simulink library "xps_library"  (Simulink 8.0)
settings: Solver=ode45  SolverMode=SingleTasking  StartTime=0.0  StopTime=10.0  RelTol=1e-3
undefined symbols (not defined in the file): sys_clk, xps_library_software_register_user_data_in
libraries: xbsIndex_r4 x867, simulink x109, dspsigops x81, casper_library_flow_control x68, xps_library x18, casper_library_misc x11
(part 7 of 10)

== system xps_library/Shared BRAM/mem ==
  note: Undo address
      | manipulation for
      | simulated data
  note: Undo data manipulation on way in and redo on way out for simulated data
  In1 : Inport
  In2 : Inport  Port=2
  In3 : Inport  Port=3
  Disregard Subsystem : xbsIndex_r4/Disregard Subsystem  Tag=discardX  block_type=disregard
  calc_add : Subsystem  mask{data_width=32, addr_width=10, sample_rate=sample_rate}
      mask prompts: data_width "data width"; addr_width "address width"; sample_rate "sample rate"
  ram : xbsIndex_r4/Single Port RAM  depth=2^addr_width  initVector=init_vals  distributed_mem=Block RAM  write_mode=Read After Write  rst=off  init_reg=0  en=off  latency=1  dbl_ovrd=off  optimize=Area  block_type=spram
  sim_addr : xbsIndex_r4/Gateway In  gui_display_data_type=Fixed-point  arith_type=Unsigned  n_bits=addr_width  bin_pt=0  preci_type=Single  exp_width=8  frac_width=24  quantization=Truncate  overflow=Wrap  period=sample_rate  dbl_ovrd=off  timing_constraint=None  locs_specified=off  LOCs={}  hdl_port=on  block_type=gatewayin
      settings: infoedit="Gateway in block.  Converts inputs of type Simulink integer, double and fixed point to  Xilinx fixed point type.<br><br>Hardware notes:  In hardware these blocks become top level input ports."  xl_area=[0, 0, 0, 0, 0, 0, 0]  sginterface={'Nallatech'=>{'xdspkit'=>{'non_memory_mapped_port'=>'sim_addr'}},'Xilinx'=>{'jtaghwcosim'=>{'non_memory_mapped_port'=>'sim_addr'},'xdspkit'=>{'non_memory_mapped_port'=>'sim_addr'}}}
  sim_data_in : xbsIndex_r4/Gateway In  gui_display_data_type=Fixed-point  arith_type=Unsigned  n_bits=32  bin_pt=0  preci_type=Single  exp_width=8  frac_width=24  quantization=Truncate  overflow=Wrap  period=sample_rate  dbl_ovrd=off  timing_constraint=None  locs_specified=off  LOCs={}  hdl_port=on  block_type=gatewayin
      settings: xl_area=[0, 0, 0, 0, 0, 0, 0]  sginterface={'Nallatech'=>{'xdspkit'=>{'non_memory_mapped_port'=>'sim_data_in'}},'Xilinx'=>{'jtaghwcosim'=>{'non_memory_mapped_port'=>'sim_data_in'},'xdspkit'=>{'non_memory_mapped_port'=>'sim_data_in'}}}
  sim_data_out : xbsIndex_r4/Gateway Out  hdl_port=on  timing_constraint=None  locs_specified=off  LOCs={'B21','B22','A22','B23','B19','C19','A20','A21','A23','B24','A24','A25','E18','D18','C18','B18'}  block_type=gatewayout
      settings: infoedit="Gateway out block.  Converts Xilinx fixed point inputs into ouputs of type Simulink integer, double, or fixed point.<P><P>Hardware notes:  In hardware these blocks become top level output ports or are discarded, depending on how they are configured."  xl_area=[0, 0, 0, 0, 0, 0, 0]  sginterface={'Nallatech'=>{'xdspkit'=>{'non_memory_mapped_port'=>'sim_data_out'}},'Xilinx'=>{'jtaghwcosim'=>{'non_memory_mapped_port'=>'sim_data_out'},'xdspkit'=>{'non_memory_mapped_port'=>'sim_data_out'}}}
  sim_munge_in : Subsystem  AncestorBlock=casper_library_flow_control/munge  mask(munge){divisions=1, div_size=32, order=[0], arith_type_out=Unsigned, bin_pt_out=0}
      mask prompts: divisions "Number of divisions"; div_size "Division size (bits)"; order "Division packing order"; arith_type_out "Output arithmetic type"; bin_pt_out "Output binary point"
      mask help: Splits an input bus into the specified number of divisions and then recombines them in the order specified (most significant division = 0,least = number divisions-1)
      mask init:
      | munge_init(gcb, ...
      |     'divisions', divisions, ...
      |     'div_size', div_size, ...
      |     'order', order, ...
      |     'arith_type_out', arith_type_out, ...
      |     'bin_pt_out', bin_pt_out);
      settings: AttributesFormatString=|
      | split:32
      | join:0
      | Unsigned [32,0]
      mask TypeOptions arith_type_out: Unsigned | Signed  (2's comp) | Floating-point
  sim_munge_out : Subsystem  AncestorBlock=casper_library_flow_control/munge  mask(munge){divisions=1, div_size=32, order=[0], arith_type_out=Unsigned, bin_pt_out=0}
      mask prompts: divisions "Number of divisions"; div_size "Division size (bits)"; order "Division packing order"; arith_type_out "Output arithmetic type"; bin_pt_out "Output binary point"
      mask help: Splits an input bus into the specified number of divisions and then recombines them in the order specified (most significant division = 0,least = number divisions-1)
      mask init:
      | munge_init(gcb, ...
      |     'divisions', divisions, ...
      |     'div_size', div_size, ...
      |     'order', order, ...
      |     'arith_type_out', arith_type_out, ...
      |     'bin_pt_out', bin_pt_out);
      settings: AttributesFormatString=|
      | split:32
      | join:0
      | Unsigned [32,0]
      mask TypeOptions arith_type_out: Unsigned | Signed  (2's comp) | Floating-point
  sim_we : xbsIndex_r4/Gateway In  gui_display_data_type=Fixed-point  arith_type=Boolean  n_bits=1  bin_pt=0  preci_type=Single  exp_width=8  frac_width=24  quantization=Truncate  overflow=Wrap  period=sample_rate  dbl_ovrd=off  timing_constraint=None  locs_specified=off  LOCs={}  hdl_port=on  block_type=gatewayin
      settings: infoedit="Gateway in block.  Converts inputs of type Simulink integer, double and fixed point to  Xilinx fixed point type.<br><br>Hardware notes:  In hardware these blocks become top level input ports."  xl_area=[0, 0, 0, 0, 0, 0, 0]  sginterface={'Nallatech'=>{'xdspkit'=>{'non_memory_mapped_port'=>'sim_we'}},'Xilinx'=>{'jtaghwcosim'=>{'non_memory_mapped_port'=>'sim_we'},'xdspkit'=>{'non_memory_mapped_port'=>'sim_we'}}}
  Out1 : Outport
  wires:
  sim_munge_in/1(dout) -> ram/2
  ram/1 -> sim_munge_out/1(din)
  sim_we/1 -> ram/3
  sim_data_in/1 -> sim_munge_in/1(din)
  sim_addr/1 -> calc_add/1(in)
  In3/1 -> sim_we/1
  sim_data_out/1 -> Out1/1
  In2/1 -> sim_data_in/1
  In1/1 -> sim_addr/1
  sim_munge_out/1(dout) -> sim_data_out/1
  calc_add/1(out) -> ram/1

== system xps_library/Shared BRAM/munge_in ==
  din : Inport
  reinterpret_out : xbsIndex_r4/Reinterpret  force_arith_type=on  arith_type=Unsigned  force_bin_pt=on  bin_pt=0  block_type=reinterpret
  dout : Outport
  wires:
  reinterpret_out/1 -> dout/1
  din/1 -> reinterpret_out/1

== system xps_library/Shared BRAM/munge_out ==
  din : Inport
  reinterpret_out : xbsIndex_r4/Reinterpret  force_arith_type=on  arith_type=Unsigned  force_bin_pt=on  bin_pt=0  block_type=reinterpret
  dout : Outport
  wires:
  reinterpret_out/1 -> dout/1
  din/1 -> reinterpret_out/1

== system xps_library/adc/conv ==
  In1 : Inport
  Concat : xbsIndex_r4/Concat  num_inputs=2  dbl_ovrd=off  block_type=concat
      settings: block_version=8.2.02
  Inverter : xbsIndex_r4/Inverter  en=off  latency=0  dbl_ovrd=off  block_type=inv
      settings: xl_area=[0, 0, 0, 0, 0, 0, 0]  block_version=8.2.02
  Reinterpret : xbsIndex_r4/Reinterpret  force_arith_type=on  arith_type="Signed  (2's comp)"  force_bin_pt=on  bin_pt=7  block_type=reinterpret
      settings: infoedit="Changes signal type without altering the binary representation.   You can changed the signal between signed and unsigned, and relocate the binary point.<P><P>Hardware notes: In hardware this block costs nothing.<P><P>Example:  Suppose the input is 6 bits wide, signed, with 2 fractional bits, and the output is forced to unsigned with 0 fractional bits.  Then an input of -2.0 (1110.00 in binary 2's complement) becomes an output of 56 (111000 in binary)."  block_version=8.2.02
  Slice : xbsIndex_r4/Slice  nbits=1  boolean_output=off  mode=Upper Bit Location + Width  bit1=0  base1=MSB of Input  bit0=0  base0=LSB of Input  dbl_ovrd=off  block_type=slice
      settings: infoedit="Extracts a given range of bits from each input sample and presents it at the output.  The output type is ordinarily unsigned with binary point at zero, but can be Boolean when the slice is one bit wide.<P><P>Hardware notes: In hardware this block costs nothing."  block_version=8.2.02
  Slice1 : xbsIndex_r4/Slice  nbits=7  boolean_output=off  mode=Lower Bit Location + Width  bit1=0  base1=MSB of Input  bit0=0  base0=LSB of Input  dbl_ovrd=off  block_type=slice
      settings: infoedit="Extracts a given range of bits from each input sample and presents it at the output.  The output type is ordinarily unsigned with binary point at zero, but can be Boolean when the slice is one bit wide.<P><P>Hardware notes: In hardware this block costs nothing."  block_version=8.2.02
  Out1 : Outport
  wires:
  Reinterpret/1 -> Out1/1
  Concat/1 -> Reinterpret/1
  Slice1/1 -> Concat/2
  Inverter/1 -> Concat/1
  Slice/1 -> Inverter/1
  In1/1 -> Slice/1, Slice1/1

== system xps_library/adc/conv1 ==
  In1 : Inport
  Concat : xbsIndex_r4/Concat  num_inputs=2  dbl_ovrd=off  block_type=concat
      settings: block_version=8.2.02
  Inverter : xbsIndex_r4/Inverter  en=off  latency=0  dbl_ovrd=off  block_type=inv
      settings: xl_area=[0, 0, 0, 0, 0, 0, 0]  block_version=8.2.02
  Reinterpret : xbsIndex_r4/Reinterpret  force_arith_type=on  arith_type="Signed  (2's comp)"  force_bin_pt=on  bin_pt=7  block_type=reinterpret
      settings: infoedit="Changes signal type without altering the binary representation.   You can changed the signal between signed and unsigned, and relocate the binary point.<P><P>Hardware notes: In hardware this block costs nothing.<P><P>Example:  Suppose the input is 6 bits wide, signed, with 2 fractional bits, and the output is forced to unsigned with 0 fractional bits.  Then an input of -2.0 (1110.00 in binary 2's complement) becomes an output of 56 (111000 in binary)."  block_version=8.2.02
  Slice : xbsIndex_r4/Slice  nbits=1  boolean_output=off  mode=Upper Bit Location + Width  bit1=0  base1=MSB of Input  bit0=0  base0=LSB of Input  dbl_ovrd=off  block_type=slice
      settings: infoedit="Extracts a given range of bits from each input sample and presents it at the output.  The output type is ordinarily unsigned with binary point at zero, but can be Boolean when the slice is one bit wide.<P><P>Hardware notes: In hardware this block costs nothing."  block_version=8.2.02
  Slice1 : xbsIndex_r4/Slice  nbits=7  boolean_output=off  mode=Lower Bit Location + Width  bit1=0  base1=MSB of Input  bit0=0  base0=LSB of Input  dbl_ovrd=off  block_type=slice
      settings: infoedit="Extracts a given range of bits from each input sample and presents it at the output.  The output type is ordinarily unsigned with binary point at zero, but can be Boolean when the slice is one bit wide.<P><P>Hardware notes: In hardware this block costs nothing."  block_version=8.2.02
  Out1 : Outport
  wires:
  Reinterpret/1 -> Out1/1
  Concat/1 -> Reinterpret/1
  Slice1/1 -> Concat/2
  Inverter/1 -> Concat/1
  Slice/1 -> Inverter/1
  In1/1 -> Slice/1, Slice1/1

== system xps_library/adc/conv2 ==
  In1 : Inport
  Concat : xbsIndex_r4/Concat  num_inputs=2  dbl_ovrd=off  block_type=concat
      settings: block_version=8.2.02
  Inverter : xbsIndex_r4/Inverter  en=off  latency=0  dbl_ovrd=off  block_type=inv
      settings: xl_area=[0, 0, 0, 0, 0, 0, 0]  block_version=8.2.02
  Reinterpret : xbsIndex_r4/Reinterpret  force_arith_type=on  arith_type="Signed  (2's comp)"  force_bin_pt=on  bin_pt=7  block_type=reinterpret
      settings: infoedit="Changes signal type without altering the binary representation.   You can changed the signal between signed and unsigned, and relocate the binary point.<P><P>Hardware notes: In hardware this block costs nothing.<P><P>Example:  Suppose the input is 6 bits wide, signed, with 2 fractional bits, and the output is forced to unsigned with 0 fractional bits.  Then an input of -2.0 (1110.00 in binary 2's complement) becomes an output of 56 (111000 in binary)."  block_version=8.2.02
  Slice : xbsIndex_r4/Slice  nbits=1  boolean_output=off  mode=Upper Bit Location + Width  bit1=0  base1=MSB of Input  bit0=0  base0=LSB of Input  dbl_ovrd=off  block_type=slice
      settings: infoedit="Extracts a given range of bits from each input sample and presents it at the output.  The output type is ordinarily unsigned with binary point at zero, but can be Boolean when the slice is one bit wide.<P><P>Hardware notes: In hardware this block costs nothing."  block_version=8.2.02
  Slice1 : xbsIndex_r4/Slice  nbits=7  boolean_output=off  mode=Lower Bit Location + Width  bit1=0  base1=MSB of Input  bit0=0  base0=LSB of Input  dbl_ovrd=off  block_type=slice
      settings: infoedit="Extracts a given range of bits from each input sample and presents it at the output.  The output type is ordinarily unsigned with binary point at zero, but can be Boolean when the slice is one bit wide.<P><P>Hardware notes: In hardware this block costs nothing."  block_version=8.2.02
  Out1 : Outport
  wires:
  Reinterpret/1 -> Out1/1
  Concat/1 -> Reinterpret/1
  Slice1/1 -> Concat/2
  Inverter/1 -> Concat/1
  Slice/1 -> Inverter/1
  In1/1 -> Slice/1, Slice1/1

== system xps_library/adc/conv3 ==
  In1 : Inport
  Concat : xbsIndex_r4/Concat  num_inputs=2  dbl_ovrd=off  block_type=concat
      settings: block_version=8.2.02
  Inverter : xbsIndex_r4/Inverter  en=off  latency=0  dbl_ovrd=off  block_type=inv
      settings: xl_area=[0, 0, 0, 0, 0, 0, 0]  block_version=8.2.02
  Reinterpret : xbsIndex_r4/Reinterpret  force_arith_type=on  arith_type="Signed  (2's comp)"  force_bin_pt=on  bin_pt=7  block_type=reinterpret
      settings: infoedit="Changes signal type without altering the binary representation.   You can changed the signal between signed and unsigned, and relocate the binary point.<P><P>Hardware notes: In hardware this block costs nothing.<P><P>Example:  Suppose the input is 6 bits wide, signed, with 2 fractional bits, and the output is forced to unsigned with 0 fractional bits.  Then an input of -2.0 (1110.00 in binary 2's complement) becomes an output of 56 (111000 in binary)."  block_version=8.2.02
  Slice : xbsIndex_r4/Slice  nbits=1  boolean_output=off  mode=Upper Bit Location + Width  bit1=0  base1=MSB of Input  bit0=0  base0=LSB of Input  dbl_ovrd=off  block_type=slice
      settings: infoedit="Extracts a given range of bits from each input sample and presents it at the output.  The output type is ordinarily unsigned with binary point at zero, but can be Boolean when the slice is one bit wide.<P><P>Hardware notes: In hardware this block costs nothing."  block_version=8.2.02
  Slice1 : xbsIndex_r4/Slice  nbits=7  boolean_output=off  mode=Lower Bit Location + Width  bit1=0  base1=MSB of Input  bit0=0  base0=LSB of Input  dbl_ovrd=off  block_type=slice
      settings: infoedit="Extracts a given range of bits from each input sample and presents it at the output.  The output type is ordinarily unsigned with binary point at zero, but can be Boolean when the slice is one bit wide.<P><P>Hardware notes: In hardware this block costs nothing."  block_version=8.2.02
  Out1 : Outport
  wires:
  Reinterpret/1 -> Out1/1
  Concat/1 -> Reinterpret/1
  Slice1/1 -> Concat/2
  Inverter/1 -> Concat/1
  Slice/1 -> Inverter/1
  In1/1 -> Slice/1, Slice1/1

== system xps_library/adc/conv4 ==
  In1 : Inport
  Concat : xbsIndex_r4/Concat  num_inputs=2  dbl_ovrd=off  block_type=concat
      settings: block_version=8.2.02
  Inverter : xbsIndex_r4/Inverter  en=off  latency=0  dbl_ovrd=off  block_type=inv
      settings: xl_area=[0, 0, 0, 0, 0, 0, 0]  block_version=8.2.02
  Reinterpret : xbsIndex_r4/Reinterpret  force_arith_type=on  arith_type="Signed  (2's comp)"  force_bin_pt=on  bin_pt=7  block_type=reinterpret
      settings: infoedit="Changes signal type without altering the binary representation.   You can changed the signal between signed and unsigned, and relocate the binary point.<P><P>Hardware notes: In hardware this block costs nothing.<P><P>Example:  Suppose the input is 6 bits wide, signed, with 2 fractional bits, and the output is forced to unsigned with 0 fractional bits.  Then an input of -2.0 (1110.00 in binary 2's complement) becomes an output of 56 (111000 in binary)."  block_version=8.2.02
  Slice : xbsIndex_r4/Slice  nbits=1  boolean_output=off  mode=Upper Bit Location + Width  bit1=0  base1=MSB of Input  bit0=0  base0=LSB of Input  dbl_ovrd=off  block_type=slice
      settings: infoedit="Extracts a given range of bits from each input sample and presents it at the output.  The output type is ordinarily unsigned with binary point at zero, but can be Boolean when the slice is one bit wide.<P><P>Hardware notes: In hardware this block costs nothing."  block_version=8.2.02
  Slice1 : xbsIndex_r4/Slice  nbits=7  boolean_output=off  mode=Lower Bit Location + Width  bit1=0  base1=MSB of Input  bit0=0  base0=LSB of Input  dbl_ovrd=off  block_type=slice
      settings: infoedit="Extracts a given range of bits from each input sample and presents it at the output.  The output type is ordinarily unsigned with binary point at zero, but can be Boolean when the slice is one bit wide.<P><P>Hardware notes: In hardware this block costs nothing."  block_version=8.2.02
  Out1 : Outport
  wires:
  Reinterpret/1 -> Out1/1
  Concat/1 -> Reinterpret/1
  Slice1/1 -> Concat/2
  Inverter/1 -> Concat/1
  Slice/1 -> Inverter/1
  In1/1 -> Slice/1, Slice1/1

== system xps_library/adc/conv5 ==
  In1 : Inport
  Concat : xbsIndex_r4/Concat  num_inputs=2  dbl_ovrd=off  block_type=concat
      settings: block_version=8.2.02
  Inverter : xbsIndex_r4/Inverter  en=off  latency=0  dbl_ovrd=off  block_type=inv
      settings: xl_area=[0, 0, 0, 0, 0, 0, 0]  block_version=8.2.02
  Reinterpret : xbsIndex_r4/Reinterpret  force_arith_type=on  arith_type="Signed  (2's comp)"  force_bin_pt=on  bin_pt=7  block_type=reinterpret
      settings: infoedit="Changes signal type without altering the binary representation.   You can changed the signal between signed and unsigned, and relocate the binary point.<P><P>Hardware notes: In hardware this block costs nothing.<P><P>Example:  Suppose the input is 6 bits wide, signed, with 2 fractional bits, and the output is forced to unsigned with 0 fractional bits.  Then an input of -2.0 (1110.00 in binary 2's complement) becomes an output of 56 (111000 in binary)."  block_version=8.2.02
  Slice : xbsIndex_r4/Slice  nbits=1  boolean_output=off  mode=Upper Bit Location + Width  bit1=0  base1=MSB of Input  bit0=0  base0=LSB of Input  dbl_ovrd=off  block_type=slice
      settings: infoedit="Extracts a given range of bits from each input sample and presents it at the output.  The output type is ordinarily unsigned with binary point at zero, but can be Boolean when the slice is one bit wide.<P><P>Hardware notes: In hardware this block costs nothing."  block_version=8.2.02
  Slice1 : xbsIndex_r4/Slice  nbits=7  boolean_output=off  mode=Lower Bit Location + Width  bit1=0  base1=MSB of Input  bit0=0  base0=LSB of Input  dbl_ovrd=off  block_type=slice
      settings: infoedit="Extracts a given range of bits from each input sample and presents it at the output.  The output type is ordinarily unsigned with binary point at zero, but can be Boolean when the slice is one bit wide.<P><P>Hardware notes: In hardware this block costs nothing."  block_version=8.2.02
  Out1 : Outport
  wires:
  Reinterpret/1 -> Out1/1
  Concat/1 -> Reinterpret/1
  Slice1/1 -> Concat/2
  Inverter/1 -> Concat/1
  Slice/1 -> Inverter/1
  In1/1 -> Slice/1, Slice1/1

== system xps_library/adc/conv6 ==
  In1 : Inport
  Concat : xbsIndex_r4/Concat  num_inputs=2  dbl_ovrd=off  block_type=concat
      settings: block_version=8.2.02
  Inverter : xbsIndex_r4/Inverter  en=off  latency=0  dbl_ovrd=off  block_type=inv
      settings: xl_area=[0, 0, 0, 0, 0, 0, 0]  block_version=8.2.02
  Reinterpret : xbsIndex_r4/Reinterpret  force_arith_type=on  arith_type="Signed  (2's comp)"  force_bin_pt=on  bin_pt=7  block_type=reinterpret
      settings: infoedit="Changes signal type without altering the binary representation.   You can changed the signal between signed and unsigned, and relocate the binary point.<P><P>Hardware notes: In hardware this block costs nothing.<P><P>Example:  Suppose the input is 6 bits wide, signed, with 2 fractional bits, and the output is forced to unsigned with 0 fractional bits.  Then an input of -2.0 (1110.00 in binary 2's complement) becomes an output of 56 (111000 in binary)."  block_version=8.2.02
  Slice : xbsIndex_r4/Slice  nbits=1  boolean_output=off  mode=Upper Bit Location + Width  bit1=0  base1=MSB of Input  bit0=0  base0=LSB of Input  dbl_ovrd=off  block_type=slice
      settings: infoedit="Extracts a given range of bits from each input sample and presents it at the output.  The output type is ordinarily unsigned with binary point at zero, but can be Boolean when the slice is one bit wide.<P><P>Hardware notes: In hardware this block costs nothing."  block_version=8.2.02
  Slice1 : xbsIndex_r4/Slice  nbits=7  boolean_output=off  mode=Lower Bit Location + Width  bit1=0  base1=MSB of Input  bit0=0  base0=LSB of Input  dbl_ovrd=off  block_type=slice
      settings: infoedit="Extracts a given range of bits from each input sample and presents it at the output.  The output type is ordinarily unsigned with binary point at zero, but can be Boolean when the slice is one bit wide.<P><P>Hardware notes: In hardware this block costs nothing."  block_version=8.2.02
  Out1 : Outport
  wires:
  Reinterpret/1 -> Out1/1
  Concat/1 -> Reinterpret/1
  Slice1/1 -> Concat/2
  Inverter/1 -> Concat/1
  Slice/1 -> Inverter/1
  In1/1 -> Slice/1, Slice1/1

== system xps_library/adc/conv7 ==
  In1 : Inport
  Concat : xbsIndex_r4/Concat  num_inputs=2  dbl_ovrd=off  block_type=concat
      settings: block_version=8.2.02
  Inverter : xbsIndex_r4/Inverter  en=off  latency=0  dbl_ovrd=off  block_type=inv
      settings: xl_area=[0, 0, 0, 0, 0, 0, 0]  block_version=8.2.02
  Reinterpret : xbsIndex_r4/Reinterpret  force_arith_type=on  arith_type="Signed  (2's comp)"  force_bin_pt=on  bin_pt=7  block_type=reinterpret
      settings: infoedit="Changes signal type without altering the binary representation.   You can changed the signal between signed and unsigned, and relocate the binary point.<P><P>Hardware notes: In hardware this block costs nothing.<P><P>Example:  Suppose the input is 6 bits wide, signed, with 2 fractional bits, and the output is forced to unsigned with 0 fractional bits.  Then an input of -2.0 (1110.00 in binary 2's complement) becomes an output of 56 (111000 in binary)."  block_version=8.2.02
  Slice : xbsIndex_r4/Slice  nbits=1  boolean_output=off  mode=Upper Bit Location + Width  bit1=0  base1=MSB of Input  bit0=0  base0=LSB of Input  dbl_ovrd=off  block_type=slice
      settings: infoedit="Extracts a given range of bits from each input sample and presents it at the output.  The output type is ordinarily unsigned with binary point at zero, but can be Boolean when the slice is one bit wide.<P><P>Hardware notes: In hardware this block costs nothing."  block_version=8.2.02
  Slice1 : xbsIndex_r4/Slice  nbits=7  boolean_output=off  mode=Lower Bit Location + Width  bit1=0  base1=MSB of Input  bit0=0  base0=LSB of Input  dbl_ovrd=off  block_type=slice
      settings: infoedit="Extracts a given range of bits from each input sample and presents it at the output.  The output type is ordinarily unsigned with binary point at zero, but can be Boolean when the slice is one bit wide.<P><P>Hardware notes: In hardware this block costs nothing."  block_version=8.2.02
  Out1 : Outport
  wires:
  Reinterpret/1 -> Out1/1
  Concat/1 -> Reinterpret/1
  Slice1/1 -> Concat/2
  Inverter/1 -> Concat/1
  Slice/1 -> Inverter/1
  In1/1 -> Slice/1, Slice1/1

== system xps_library/adc083000x2/adc_sim ==
  sim_adc_data_in : Inport
  adc_bias : Bias  Bias=128  SaturateOnIntegerOverflow=on
  adc_gain : Gain  Gain=128
  overflow_detector : Subsystem  AncestorBlock=casper_library/Misc/of_detect_bus  mask(of_detect_bus){nStreams=16, bit_width=8}
      mask prompts: nStreams "Number of Streams"; bit_width "Bit Width"
      mask init:
      | adc_overflow_detector_init(gcb, ...
      |     'nStreams', nStreams, ...
      |     'bit_width', bit_width);
  sample0_ds : dspsigops/Downsample  N=16  phase=1  smode=Force single rate  fmode=Maintain input frame rate  ic=0
  sample10_ds : dspsigops/Downsample  N=16  phase=11  smode=Force single rate  fmode=Maintain input frame rate  ic=0
  sample11_ds : dspsigops/Downsample  N=16  phase=12  smode=Force single rate  fmode=Maintain input frame rate  ic=0
  sample12_ds : dspsigops/Downsample  N=16  phase=13  smode=Force single rate  fmode=Maintain input frame rate  ic=0
  sample13_ds : dspsigops/Downsample  N=16  phase=14  smode=Force single rate  fmode=Maintain input frame rate  ic=0
  sample14_ds : dspsigops/Downsample  N=16  phase=15  smode=Force single rate  fmode=Maintain input frame rate  ic=0
  sample15_ds : dspsigops/Downsample  N=16  phase=0  smode=Force single rate  fmode=Maintain input frame rate  ic=0
  sample1_ds : dspsigops/Downsample  N=16  phase=2  smode=Force single rate  fmode=Maintain input frame rate  ic=0
  sample2_ds : dspsigops/Downsample  N=16  phase=3  smode=Force single rate  fmode=Maintain input frame rate  ic=0
  sample3_ds : dspsigops/Downsample  N=16  phase=4  smode=Force single rate  fmode=Maintain input frame rate  ic=0
  sample4_ds : dspsigops/Downsample  N=16  phase=5  smode=Force single rate  fmode=Maintain input frame rate  ic=0
  sample5_ds : dspsigops/Downsample  N=16  phase=6  smode=Force single rate  fmode=Maintain input frame rate  ic=0
  sample6_ds : dspsigops/Downsample  N=16  phase=7  smode=Force single rate  fmode=Maintain input frame rate  ic=0
  sample7_ds : dspsigops/Downsample  N=16  phase=8  smode=Force single rate  fmode=Maintain input frame rate  ic=0
  sample8_ds : dspsigops/Downsample  N=16  phase=9  smode=Force single rate  fmode=Maintain input frame rate  ic=0
  sample9_ds : dspsigops/Downsample  N=16  phase=10  smode=Force single rate  fmode=Maintain input frame rate  ic=0
  s0 : Outport
  s1 : Outport  Port=2
  s2 : Outport  Port=3
  s3 : Outport  Port=4
  s4 : Outport  Port=5
  s5 : Outport  Port=6
  s6 : Outport  Port=7
  s7 : Outport  Port=8
  s8 : Outport  Port=9
  s9 : Outport  Port=10
  s10 : Outport  Port=11
  s11 : Outport  Port=12
  s12 : Outport  Port=13
  s13 : Outport  Port=14
  s14 : Outport  Port=15
  s15 : Outport  Port=16
  of : Outport  Port=17
  wires:
  sim_adc_data_in/1 -> adc_gain/1
  adc_gain/1 -> adc_bias/1
  overflow_detector/1(overflow) -> of/1
  adc_bias/1 -> sample0_ds/1, sample1_ds/1, sample2_ds/1, sample3_ds/1, sample4_ds/1, sample5_ds/1, sample6_ds/1, sample7_ds/1, sample8_ds/1, sample9_ds/1, sample10_ds/1, sample11_ds/1, sample12_ds/1, sample13_ds/1, sample14_ds/1, sample15_ds/1
  sample0_ds/1 -> overflow_detector/1(s0), s0/1
  sample1_ds/1 -> overflow_detector/2(s1), s1/1
  sample2_ds/1 -> overflow_detector/3(s2), s2/1
  sample3_ds/1 -> overflow_detector/4(s3), s3/1
  sample4_ds/1 -> overflow_detector/5(s4), s4/1
  sample5_ds/1 -> overflow_detector/6(s5), s5/1
  sample6_ds/1 -> overflow_detector/7(s6), s6/1
  sample7_ds/1 -> overflow_detector/8(s7), s7/1
  sample8_ds/1 -> overflow_detector/9(s8), s8/1
  sample9_ds/1 -> overflow_detector/10(s9), s9/1
  sample10_ds/1 -> overflow_detector/11(s10), s10/1
  sample11_ds/1 -> overflow_detector/12(s11), s11/1
  sample12_ds/1 -> overflow_detector/13(s12), s12/1
  sample13_ds/1 -> overflow_detector/14(s13), s13/1
  sample14_ds/1 -> overflow_detector/15(s14), s14/1
  sample15_ds/1 -> overflow_detector/16(s15), s15/1

== system xps_library/adc1x1800-10/conv ==
  In1 : Inport
  Concat : xbsIndex_r4/Concat  num_inputs=2  dbl_ovrd=off  block_type=concat
      settings: block_version=8.2.02
  Inverter : xbsIndex_r4/Inverter  en=off  latency=0  dbl_ovrd=off  block_type=inv
      settings: xl_area=[0, 0, 0, 0, 0, 0, 0]  block_version=8.2.02
  Reinterpret : xbsIndex_r4/Reinterpret  force_arith_type=on  arith_type="Signed  (2's comp)"  force_bin_pt=on  bin_pt=9  block_type=reinterpret
      settings: infoedit="Changes signal type without altering the binary representation.   You can changed the signal between signed and unsigned, and relocate the binary point.<br><br>Hardware notes: In hardware this block costs nothing.<br><br>Example:  Suppose the input is 6 bits wide, signed, with 2 fractional bits, and the output is forced to unsigned with 0 fractional bits.  Then an input of -2.0 (1110.00 in binary 2's complement) becomes an output of 56 (111000 in binary)."  block_version=8.2.02
  Slice : xbsIndex_r4/Slice  nbits=1  boolean_output=off  mode=Upper Bit Location + Width  bit1=0  base1=MSB of Input  bit0=0  base0=LSB of Input  dbl_ovrd=off  block_type=slice
      settings: block_version=8.2.02
  Slice1 : xbsIndex_r4/Slice  nbits=9  boolean_output=off  mode=Lower Bit Location + Width  bit1=0  base1=MSB of Input  bit0=0  base0=LSB of Input  dbl_ovrd=off  block_type=slice
      settings: block_version=8.2.02
  Out1 : Outport
  wires:
  In1/1 -> Slice1/1, Slice/1
  Slice/1 -> Inverter/1
  Inverter/1 -> Concat/1
  Slice1/1 -> Concat/2
  Concat/1 -> Reinterpret/1
  Reinterpret/1 -> Out1/1

== system xps_library/adc1x1800-10/conv1 ==
  In1 : Inport
  Concat : xbsIndex_r4/Concat  num_inputs=2  dbl_ovrd=off  block_type=concat
      settings: block_version=8.2.02
  Inverter : xbsIndex_r4/Inverter  en=off  latency=0  dbl_ovrd=off  block_type=inv
      settings: xl_area=[0, 0, 0, 0, 0, 0, 0]  block_version=8.2.02
  Reinterpret : xbsIndex_r4/Reinterpret  force_arith_type=on  arith_type="Signed  (2's comp)"  force_bin_pt=on  bin_pt=9  block_type=reinterpret
      settings: infoedit="Changes signal type without altering the binary representation.   You can changed the signal between signed and unsigned, and relocate the binary point.<br><br>Hardware notes: In hardware this block costs nothing.<br><br>Example:  Suppose the input is 6 bits wide, signed, with 2 fractional bits, and the output is forced to unsigned with 0 fractional bits.  Then an input of -2.0 (1110.00 in binary 2's complement) becomes an output of 56 (111000 in binary)."  block_version=8.2.02
  Slice : xbsIndex_r4/Slice  nbits=1  boolean_output=off  mode=Upper Bit Location + Width  bit1=0  base1=MSB of Input  bit0=0  base0=LSB of Input  dbl_ovrd=off  block_type=slice
      settings: block_version=8.2.02
  Slice1 : xbsIndex_r4/Slice  nbits=9  boolean_output=off  mode=Lower Bit Location + Width  bit1=0  base1=MSB of Input  bit0=0  base0=LSB of Input  dbl_ovrd=off  block_type=slice
      settings: block_version=8.2.02
  Out1 : Outport
  wires:
  In1/1 -> Slice1/1, Slice/1
  Slice/1 -> Inverter/1
  Inverter/1 -> Concat/1
  Slice1/1 -> Concat/2
  Concat/1 -> Reinterpret/1
  Reinterpret/1 -> Out1/1

== system xps_library/adc1x1800-10/conv2 ==
  In1 : Inport
  Concat : xbsIndex_r4/Concat  num_inputs=2  dbl_ovrd=off  block_type=concat
      settings: block_version=8.2.02
  Inverter : xbsIndex_r4/Inverter  en=off  latency=0  dbl_ovrd=off  block_type=inv
      settings: xl_area=[0, 0, 0, 0, 0, 0, 0]  block_version=8.2.02
  Reinterpret : xbsIndex_r4/Reinterpret  force_arith_type=on  arith_type="Signed  (2's comp)"  force_bin_pt=on  bin_pt=9  block_type=reinterpret
      settings: infoedit="Changes signal type without altering the binary representation.   You can changed the signal between signed and unsigned, and relocate the binary point.<br><br>Hardware notes: In hardware this block costs nothing.<br><br>Example:  Suppose the input is 6 bits wide, signed, with 2 fractional bits, and the output is forced to unsigned with 0 fractional bits.  Then an input of -2.0 (1110.00 in binary 2's complement) becomes an output of 56 (111000 in binary)."  block_version=8.2.02
  Slice : xbsIndex_r4/Slice  nbits=1  boolean_output=off  mode=Upper Bit Location + Width  bit1=0  base1=MSB of Input  bit0=0  base0=LSB of Input  dbl_ovrd=off  block_type=slice
      settings: block_version=8.2.02
  Slice1 : xbsIndex_r4/Slice  nbits=9  boolean_output=off  mode=Lower Bit Location + Width  bit1=0  base1=MSB of Input  bit0=0  base0=LSB of Input  dbl_ovrd=off  block_type=slice
      settings: block_version=8.2.02
  Out1 : Outport
  wires:
  In1/1 -> Slice1/1, Slice/1
  Slice/1 -> Inverter/1
  Inverter/1 -> Concat/1
  Slice1/1 -> Concat/2
  Concat/1 -> Reinterpret/1
  Reinterpret/1 -> Out1/1

== system xps_library/adc1x1800-10/conv3 ==
  In1 : Inport
  Concat : xbsIndex_r4/Concat  num_inputs=2  dbl_ovrd=off  block_type=concat
      settings: block_version=8.2.02
  Inverter : xbsIndex_r4/Inverter  en=off  latency=0  dbl_ovrd=off  block_type=inv
      settings: xl_area=[0, 0, 0, 0, 0, 0, 0]  block_version=8.2.02
  Reinterpret : xbsIndex_r4/Reinterpret  force_arith_type=on  arith_type="Signed  (2's comp)"  force_bin_pt=on  bin_pt=9  block_type=reinterpret
      settings: infoedit="Changes signal type without altering the binary representation.   You can changed the signal between signed and unsigned, and relocate the binary point.<br><br>Hardware notes: In hardware this block costs nothing.<br><br>Example:  Suppose the input is 6 bits wide, signed, with 2 fractional bits, and the output is forced to unsigned with 0 fractional bits.  Then an input of -2.0 (1110.00 in binary 2's complement) becomes an output of 56 (111000 in binary)."  block_version=8.2.02
  Slice : xbsIndex_r4/Slice  nbits=1  boolean_output=off  mode=Upper Bit Location + Width  bit1=0  base1=MSB of Input  bit0=0  base0=LSB of Input  dbl_ovrd=off  block_type=slice
      settings: block_version=8.2.02
  Slice1 : xbsIndex_r4/Slice  nbits=9  boolean_output=off  mode=Lower Bit Location + Width  bit1=0  base1=MSB of Input  bit0=0  base0=LSB of Input  dbl_ovrd=off  block_type=slice
      settings: block_version=8.2.02
  Out1 : Outport
  wires:
  In1/1 -> Slice1/1, Slice/1
  Slice/1 -> Inverter/1
  Inverter/1 -> Concat/1
  Slice1/1 -> Concat/2
  Concat/1 -> Reinterpret/1
  Reinterpret/1 -> Out1/1

== system xps_library/adc1x1800-10/conv4 ==
  In1 : Inport
  Concat : xbsIndex_r4/Concat  num_inputs=2  dbl_ovrd=off  block_type=concat
      settings: block_version=8.2.02
  Inverter : xbsIndex_r4/Inverter  en=off  latency=0  dbl_ovrd=off  block_type=inv
      settings: xl_area=[0, 0, 0, 0, 0, 0, 0]  block_version=8.2.02
  Reinterpret : xbsIndex_r4/Reinterpret  force_arith_type=on  arith_type="Signed  (2's comp)"  force_bin_pt=on  bin_pt=9  block_type=reinterpret
      settings: infoedit="Changes signal type without altering the binary representation.   You can changed the signal between signed and unsigned, and relocate the binary point.<br><br>Hardware notes: In hardware this block costs nothing.<br><br>Example:  Suppose the input is 6 bits wide, signed, with 2 fractional bits, and the output is forced to unsigned with 0 fractional bits.  Then an input of -2.0 (1110.00 in binary 2's complement) becomes an output of 56 (111000 in binary)."  block_version=8.2.02
  Slice : xbsIndex_r4/Slice  nbits=1  boolean_output=off  mode=Upper Bit Location + Width  bit1=0  base1=MSB of Input  bit0=0  base0=LSB of Input  dbl_ovrd=off  block_type=slice
      settings: block_version=8.2.02
  Slice1 : xbsIndex_r4/Slice  nbits=9  boolean_output=off  mode=Lower Bit Location + Width  bit1=0  base1=MSB of Input  bit0=0  base0=LSB of Input  dbl_ovrd=off  block_type=slice
      settings: block_version=8.2.02
  Out1 : Outport
  wires:
  In1/1 -> Slice1/1, Slice/1
  Slice/1 -> Inverter/1
  Inverter/1 -> Concat/1
  Slice1/1 -> Concat/2
  Concat/1 -> Reinterpret/1
  Reinterpret/1 -> Out1/1

== system xps_library/adc1x1800-10/conv5 ==
  In1 : Inport
  Concat : xbsIndex_r4/Concat  num_inputs=2  dbl_ovrd=off  block_type=concat
      settings: block_version=8.2.02
  Inverter : xbsIndex_r4/Inverter  en=off  latency=0  dbl_ovrd=off  block_type=inv
      settings: xl_area=[0, 0, 0, 0, 0, 0, 0]  block_version=8.2.02
  Reinterpret : xbsIndex_r4/Reinterpret  force_arith_type=on  arith_type="Signed  (2's comp)"  force_bin_pt=on  bin_pt=9  block_type=reinterpret
      settings: infoedit="Changes signal type without altering the binary representation.   You can changed the signal between signed and unsigned, and relocate the binary point.<br><br>Hardware notes: In hardware this block costs nothing.<br><br>Example:  Suppose the input is 6 bits wide, signed, with 2 fractional bits, and the output is forced to unsigned with 0 fractional bits.  Then an input of -2.0 (1110.00 in binary 2's complement) becomes an output of 56 (111000 in binary)."  block_version=8.2.02
  Slice : xbsIndex_r4/Slice  nbits=1  boolean_output=off  mode=Upper Bit Location + Width  bit1=0  base1=MSB of Input  bit0=0  base0=LSB of Input  dbl_ovrd=off  block_type=slice
      settings: block_version=8.2.02
  Slice1 : xbsIndex_r4/Slice  nbits=9  boolean_output=off  mode=Lower Bit Location + Width  bit1=0  base1=MSB of Input  bit0=0  base0=LSB of Input  dbl_ovrd=off  block_type=slice
      settings: block_version=8.2.02
  Out1 : Outport
  wires:
  In1/1 -> Slice1/1, Slice/1
  Slice/1 -> Inverter/1
  Inverter/1 -> Concat/1
  Slice1/1 -> Concat/2
  Concat/1 -> Reinterpret/1
  Reinterpret/1 -> Out1/1

== system xps_library/adc1x1800-10/conv6 ==
  In1 : Inport
  Concat : xbsIndex_r4/Concat  num_inputs=2  dbl_ovrd=off  block_type=concat
      settings: block_version=8.2.02
  Inverter : xbsIndex_r4/Inverter  en=off  latency=0  dbl_ovrd=off  block_type=inv
      settings: xl_area=[0, 0, 0, 0, 0, 0, 0]  block_version=8.2.02
  Reinterpret : xbsIndex_r4/Reinterpret  force_arith_type=on  arith_type="Signed  (2's comp)"  force_bin_pt=on  bin_pt=9  block_type=reinterpret
      settings: infoedit="Changes signal type without altering the binary representation.   You can changed the signal between signed and unsigned, and relocate the binary point.<br><br>Hardware notes: In hardware this block costs nothing.<br><br>Example:  Suppose the input is 6 bits wide, signed, with 2 fractional bits, and the output is forced to unsigned with 0 fractional bits.  Then an input of -2.0 (1110.00 in binary 2's complement) becomes an output of 56 (111000 in binary)."  block_version=8.2.02
  Slice : xbsIndex_r4/Slice  nbits=1  boolean_output=off  mode=Upper Bit Location + Width  bit1=0  base1=MSB of Input  bit0=0  base0=LSB of Input  dbl_ovrd=off  block_type=slice
      settings: block_version=8.2.02
  Slice1 : xbsIndex_r4/Slice  nbits=9  boolean_output=off  mode=Lower Bit Location + Width  bit1=0  base1=MSB of Input  bit0=0  base0=LSB of Input  dbl_ovrd=off  block_type=slice
      settings: block_version=8.2.02
  Out1 : Outport
  wires:
  In1/1 -> Slice1/1, Slice/1
  Slice/1 -> Inverter/1
  Inverter/1 -> Concat/1
  Slice1/1 -> Concat/2
  Concat/1 -> Reinterpret/1
  Reinterpret/1 -> Out1/1

== system xps_library/adc1x1800-10/conv7 ==
  In1 : Inport
  Concat : xbsIndex_r4/Concat  num_inputs=2  dbl_ovrd=off  block_type=concat
      settings: block_version=8.2.02
  Inverter : xbsIndex_r4/Inverter  en=off  latency=0  dbl_ovrd=off  block_type=inv
      settings: xl_area=[0, 0, 0, 0, 0, 0, 0]  block_version=8.2.02
  Reinterpret : xbsIndex_r4/Reinterpret  force_arith_type=on  arith_type="Signed  (2's comp)"  force_bin_pt=on  bin_pt=9  block_type=reinterpret
      settings: infoedit="Changes signal type without altering the binary representation.   You can changed the signal between signed and unsigned, and relocate the binary point.<br><br>Hardware notes: In hardware this block costs nothing.<br><br>Example:  Suppose the input is 6 bits wide, signed, with 2 fractional bits, and the output is forced to unsigned with 0 fractional bits.  Then an input of -2.0 (1110.00 in binary 2's complement) becomes an output of 56 (111000 in binary)."  block_version=8.2.02
  Slice : xbsIndex_r4/Slice  nbits=1  boolean_output=off  mode=Upper Bit Location + Width  bit1=0  base1=MSB of Input  bit0=0  base0=LSB of Input  dbl_ovrd=off  block_type=slice
      settings: block_version=8.2.02
  Slice1 : xbsIndex_r4/Slice  nbits=9  boolean_output=off  mode=Lower Bit Location + Width  bit1=0  base1=MSB of Input  bit0=0  base0=LSB of Input  dbl_ovrd=off  block_type=slice
      settings: block_version=8.2.02
  Out1 : Outport
  wires:
  In1/1 -> Slice1/1, Slice/1
  Slice/1 -> Inverter/1
  Inverter/1 -> Concat/1
  Slice1/1 -> Concat/2
  Concat/1 -> Reinterpret/1
  Reinterpret/1 -> Out1/1
